simulink library "Geartrain_Lib"  (R2025a)
settings: Solver=ode45  StartTime=0.0  StopTime=10.0  RelTol=1e-3  EnableMultiTasking=on
undefined symbols (not defined in the file): WT_Params
libraries: fl_lib x8, sdl_lib x3, nesl_utility x2, Brakes_Lib x1
Description:
  | Copyright 2009-2025 The MathWorks, Inc. MathWorks, Inc.
settings Model: Creator=smiller  LastModifiedBy=smiller
settings SolverCC: AlgebraicLoopSolver=TrustRegion
settings DataIOCC: LimitDataPoints=on  SaveFormat=Array  SignalLoggingSaveFormat=ModelDataLogs  ReturnWorkspaceOutputs=off
settings OptimizationCC: ReuseModelBlockBuffer=off  ExpressionDepthLimit=2147483647.0  LifeSpan=inf
settings DebuggingCC: UnderspecifiedInitializationDetection=Classic  MergeDetectMultiDrivingBlocksExec=none  SolverPrmCheckMsg=warning  FcnCallInpInsideContextMsg=warning  UnconnectedInputMsg=warning  UnconnectedOutputMsg=warning  UnconnectedLineMsg=warning  AllowSymbolicDim=off  StateNameClashWarn=warning  PregeneratedLibrarySubsystemCodeDiagnostic=none  SFUnexpectedBacktrackingDiag=warning  SFNoUnconditionalDefaultTransitionDiag=warning  SFExecutionAtInitializationDiag=none  ArithmeticOperatorsInVariantConditions=warning
settings HardwareCC: ProdBitPerPointer=32.0  ProdBitPerSizeT=32.0  ProdBitPerPtrDiffT=32.0  ProdLargestAtomicFloat=None  ProdIntDivRoundTo=Undefined  ProdEndianess=Unspecified  ProdWordSize=32.0  ProdHWDeviceType=32-bit Generic
settings ModelReferenceCC: EnableRefExpFcnMdlSchedulingChecks=on  PropagateSignalLabelsOutOfModel=off
settings SFSimCC: SimUseLocalCustomCode=off  CustomCodeUndefinedFunction=UseInterfaceOnly
settings RTWCC: RTWUseLocalCustomCode=off  GPUComputeCapability=3.5  DLArmComputeVersion=19.05
settings CodeAppCC: StateflowObjectComments=on
settings GRTTargetCC: TargetLangStandard=C89/C90 (ANSI)  CombineOutputUpdateFcns=off  GRTInterface=on
settings ConfigComp: CovMetricSettings=dw  CovSaveCumulativeToWorkspaceVar=on  CovSaveSingleToWorkspaceVar=on  CovExternalEMLEnable=off  CovSFcnEnable=off

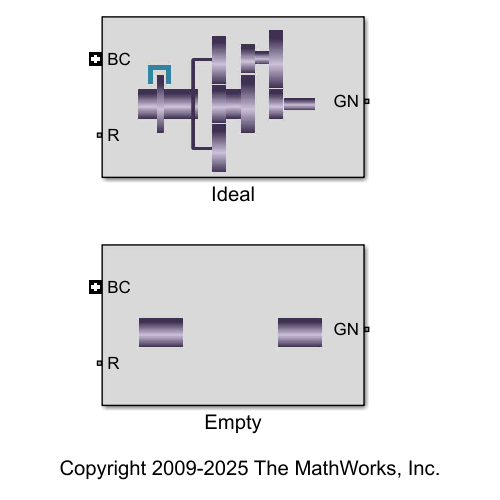
[thumbnail: Simulink's stored preview of the top-level diagram]
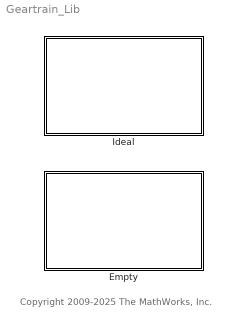
== system Geartrain_Lib ==
  note: Copyright 2009-2025 The MathWorks, Inc.
  Empty : Subsystem
      mask Display: image('Geartrain_Empty_IMAGE.jpg');
  Ideal : Subsystem
      mask Display: image('Geartrain_Ideal_IMAGE.jpg');

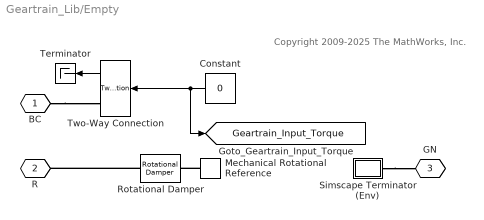
== system Geartrain_Lib/Empty ==
  note: Copyright 2009-2025 The MathWorks, Inc.
  Constant : Constant  Value=0
  Mechanical Rotational Reference : fl_lib/Mechanical/Rotational Elements/Mechanical Rotational Reference
  Rotational Damper : fl_lib/Mechanical/Rotational Elements/Rotational Damper  D=WT_Params.Empty_Geartrain.damping N*m/(rad/s)  w_specify=off  w_priority=High  w=0 rad/s  w_nominal_specify=off  w_nominal_value=1  w_nominal_unit=rad/s  t_specify=off  t_priority=High  t=0 N*m  t_nominal_specify=off  t_nominal_value=1  t_nominal_unit=N*m
  Simscape Terminator (Env) : Subsystem
      mask Display:
      | plot([0 0.9],[0.5 0.5]);
      | plot([0.5 0.9],[0.3 0.3]);
      | plot([0.5 0.9],[0.7 0.7]);
      | plot([0.9 0.9],[0.7 0.3]);
  Terminator : Terminator
  Two-Way Connection : TwoWayConnection
  BC : PMIOPort  Tag=PMCPort  Side=Left
  R : PMIOPort  Tag=PMCPort  Port=2  Side=Left
  GN : PMIOPort  Tag=PMCPort  Port=3  Side=Right
  tag scope: Geartrain_Input_Torque=global
  wires:
  Two-Way Connection/1 -> Terminator/1
  Constant/1 -> Two-Way Connection/1, [Geartrain_Input_Torque]
  connections:
  BC/RConn1 -- Two-Way Connection/RConn1
  Simscape Terminator (Env)/LConn1 -- GN/RConn1
  Rotational Damper/LConn1 -- R/RConn1
  Mechanical Rotational Reference/LConn1 -- Rotational Damper/RConn1

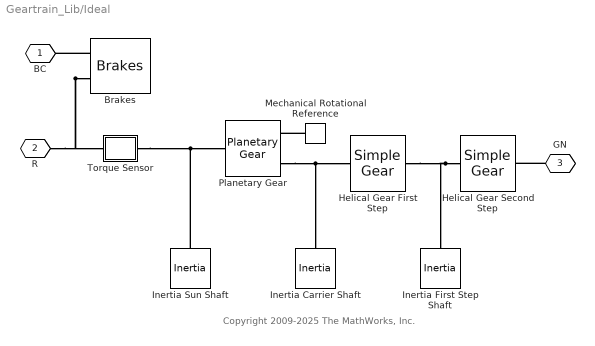
== system Geartrain_Lib/Ideal ==
  note: Copyright 2009-2025 The MathWorks, Inc.
  Brakes : Brakes_Lib/Brakes  SystemSampleTime=-1  VariantActivationTime=update diagram  EmptyChoice=off  PassThrough=off  PassThroughVariantControl=(default)  EmptyChoiceVariantControl=(default)  AllowFlexibleInterface=on  Latency=0  AutoFrameSizeCalculation=off
  Helical Gear First Step : sdl_lib/Gears/Simple Gear  ratio=WT_Params.Geartrain.Gear_Ratio.first_step  rotation_direction=3-2*(2)  friction_model=1  T_noload=0.1 N*m  T_nom=5 N*m  efficiency_nom=0.8  efficiency=0.8  temperature_TLU=[ 280 300 320 ] K  load_TLU=[ 1 5 10 ] N*m  efficiency_TLU=[ 0.95 0.9 0.85 ]  efficiency_TLU2=[ 0.85 0.8 0.75; 0.95 0.9 0.85; 0.85 0.8 0.7 ]  w_thr=0.01 rad/s  pwr_thr=0.001 W  enable_backlash=false  hardstop_model=simscape.enum.hardstop.smooth  backlash_distance=1e-3 mm  r_base=0.1 m  transition=1e-4 mm  backlash_stiffness=1e7 N/m  backlash_damping=1e6 N*s/m  coeff_rest=0  v_tol=0.001 m/s  f_tol=0 N  mu_visc=[ 0 0 ] N*m/(rad/s)  thermal_mass=50 J/K  temperature_specify=off  temperature_priority=High  temperature=300 K  temperature_nominal_specify=off  temperature_nominal_value=1  temperature_nominal_unit=K  x_backlash_specify=off  x_backlash_priority=None  x_backlash=0 mm  x_backlash_nominal_specify=off  x_backlash_nominal_value=1  x_backlash_nominal_unit=mm  f_hardstop_specify=off  f_hardstop_priority=None  f_hardstop=0 N  f_hardstop_nominal_specify=off  f_hardstop_nominal_value=1  f_hardstop_nominal_unit=N  v_backlash_specify=off  v_backlash_priority=None  v_backlash=0 m/s  v_backlash_nominal_specify=off  v_backlash_nominal_value=1  v_backlash_nominal_unit=m/s
  Helical Gear Second Step : sdl_lib/Gears/Simple Gear  ratio=WT_Params.Geartrain.Gear_Ratio.second_step_primary_generator  rotation_direction=3-2*(2)  friction_model=1  T_noload=0.1 N*m  T_nom=5 N*m  efficiency_nom=0.8  efficiency=0.8  temperature_TLU=[ 280 300 320 ] K  load_TLU=[ 1 5 10 ] N*m  efficiency_TLU=[ 0.95 0.9 0.85 ]  efficiency_TLU2=[ 0.85 0.8 0.75; 0.95 0.9 0.85; 0.85 0.8 0.7 ]  w_thr=0.01 rad/s  pwr_thr=0.001 W  enable_backlash=false  hardstop_model=simscape.enum.hardstop.smooth  backlash_distance=1e-3 mm  r_base=0.1 m  transition=1e-4 mm  backlash_stiffness=1e7 N/m  backlash_damping=1e6 N*s/m  coeff_rest=0  v_tol=0.001 m/s  f_tol=0 N  mu_visc=[ 0 0 ] N*m/(rad/s)  thermal_mass=50 J/K  temperature_specify=off  temperature_priority=High  temperature=300 K  temperature_nominal_specify=off  temperature_nominal_value=1  temperature_nominal_unit=K  x_backlash_specify=off  x_backlash_priority=None  x_backlash=0 mm  x_backlash_nominal_specify=off  x_backlash_nominal_value=1  x_backlash_nominal_unit=mm  f_hardstop_specify=off  f_hardstop_priority=None  f_hardstop=0 N  f_hardstop_nominal_specify=off  f_hardstop_nominal_value=1  f_hardstop_nominal_unit=N  v_backlash_specify=off  v_backlash_priority=None  v_backlash=0 m/s  v_backlash_nominal_specify=off  v_backlash_nominal_value=1  v_backlash_nominal_unit=m/s
  Inertia Carrier Shaft : fl_lib/Mechanical/Rotational Elements/Inertia  inertia=WT_Params.Geartrain.inertia_sun_shaft kg*m^2  num_ports=foundation.enum.numPorts2.one  w_specify=on  w_priority=High  w=0 rad/s  w_nominal_specify=off  w_nominal_value=1  w_nominal_unit=rad/s  t_specify=off  t_priority=High  t=0 N*m  t_nominal_specify=off  t_nominal_value=1  t_nominal_unit=N*m
  Inertia First Step Shaft : fl_lib/Mechanical/Rotational Elements/Inertia  inertia=WT_Params.Geartrain.inertia_first_step_shaft kg*m^2  num_ports=foundation.enum.numPorts2.one  w_specify=on  w_priority=High  w=0 rad/s  w_nominal_specify=off  w_nominal_value=1  w_nominal_unit=rad/s  t_specify=off  t_priority=High  t=0 N*m  t_nominal_specify=off  t_nominal_value=1  t_nominal_unit=N*m
  Inertia Sun Shaft : fl_lib/Mechanical/Rotational Elements/Inertia  inertia=WT_Params.Geartrain.inertia_sun_shaft kg*m^2  num_ports=foundation.enum.numPorts2.one  w_specify=on  w_priority=High  w=0 rad/s  w_nominal_specify=off  w_nominal_value=1  w_nominal_unit=rad/s  t_specify=off  t_priority=High  t=0 N*m  t_nominal_specify=off  t_nominal_value=1  t_nominal_unit=N*m
  Mechanical Rotational Reference : fl_lib/Mechanical/Rotational Elements/Mechanical Rotational Reference
  Planetary Gear : sdl_lib/Gears/Planetary Gear  rs_ratio=WT_Params.Geartrain.Gear_Ratio.planetary  friction_model=1  efficiency=[ 0.96 0.98 ]  temperature_TLU=[ 280 300 320 ] K  efficiency_sp_TLU=[ 0.95 0.9 0.85 ]  efficiency_rp_TLU=[ 0.95 0.9 0.85 ]  pwr_thr=[ 0.001 0.001 ] W  mu_visc=WT_Params.Geartrain.Planetary.viscous_losses N*m/(rad/s)  model_inertia=0  sun_inertia=1e-10 kg*m^2  ring_inertia=1e-10 kg*m^2  carrier_inertia=1e-10 kg*m^2  carrier_radius=0.01 m  planet_inertia=0.001 kg*m^2  planet_mass=1e-10 kg  thermal_mass=50 J/K  T_init=300 K
  Torque Sensor : Subsystem
      mask Display: disp('S');
  BC : PMIOPort  Tag=PMCPort  Side=Left
  R : PMIOPort  Tag=PMCPort  Port=2  Side=Left
  GN : PMIOPort  Tag=PMCPort  Port=3  Side=Right
  connections:
  Planetary Gear/RConn2 -- Helical Gear First Step/RConn1 -- Inertia Carrier Shaft/LConn1
  Helical Gear Second Step/RConn1 -- Helical Gear First Step/LConn1 -- Inertia First Step Shaft/LConn1
  Inertia Sun Shaft/LConn1 -- Planetary Gear/LConn1 -- Torque Sensor/RConn1
  Mechanical Rotational Reference/LConn1 -- Planetary Gear/RConn1
  Brakes/LConn2 -- R/RConn1 -- Torque Sensor/LConn1
  Brakes/LConn1 -- BC/RConn1
  GN/RConn1 -- Helical Gear Second Step/LConn1

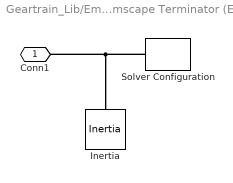
== system Geartrain_Lib/Empty/Simscape Terminator (Env) ==
  Inertia : fl_lib/Mechanical/Rotational Elements/Inertia  inertia=1.5e-3 kg*m^2  num_ports=foundation.enum.numPorts2.one  w_specify=on  w_priority=High  w=0 rad/s  w_nominal_specify=off  w_nominal_value=1  w_nominal_unit=rad/s  t_specify=off  t_priority=High  t=0 N*m  t_nominal_specify=off  t_nominal_value=1  t_nominal_unit=N*m
  Solver Configuration : nesl_utility/Solver Configuration  PhysicalDomain=network_engine_domain  SubClassName=solver  LeftPortType=input  RightPortType=generic  Tones=[]  Harmonics=[]  SimulateNoise=off  Profile=off  UseLocalSampling=off  EnableSwitchedLinearOptims=on  FrequencyDomain=off  UseCCode=off  RelTol=0.001  AbsTol=1e-06  MinStep=1e-09  ToWorkspace=off  RevertToSquareIcSolve=off  NumHomotopyIterations=100  PhasorMode=off  PhasorModeNumHarmonics=1  ConsistencySolver=NEWTON_FTOL  IndexReductionMethod=DerivativeReplacement  DoDC=off  ResidualTolerance=1e-9  ConsistencyTolSource=GLOBAL  ConsistencyAbsTol=0.001  ConsistencyRelTol=0.001  ConsistencyTolFactor=0.001  UseLocalSolver=off  LocalSolverChoice=NE_BACKWARD_EULER_ADVANCER  ResolveIndetEquations=on  FunctionEvalNumThread=1  LocalSolverSampleTime=.001  DoFixedCost=off  MaxNonlinIter=3  MaxModeIter=2  ComputeImpulses=off  ImpulseIterations=2  LinearAlgebra=Sparse  LinearAlgebraNumThread=0  EquationFormulation=NE_TIME_EF  DelaysMemoryBudget=1024  AutomaticFiltering=on  FilteringTimeConstant=0.001  PartitionStorageMethod=AS_NEEDED  PartitionMemoryBudget=1024  PartitionMethod=FAST  MultibodyUseLocalSolver=off  MultibodyLocalSolverChoice=ODE1  MultibodyLocalSolverSampleTime=0.001
  Conn1 : PMIOPort  Side=Left
  connections:
  Solver Configuration/RConn1 -- Conn1/RConn1 -- Inertia/LConn1

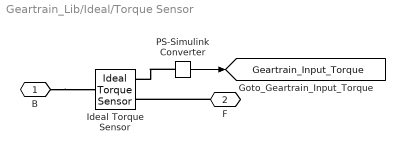
== system Geartrain_Lib/Ideal/Torque Sensor ==
  Ideal Torque Sensor : fl_lib/Mechanical/Mechanical Sensors/Ideal Torque Sensor
  PS-Simulink Converter : nesl_utility/PS-Simulink Converter  PhysicalDomain=network_engine_domain  SubClassName=ps_output  LeftPortType=input  RightPortType=output  PseudoPeriodic=off  Frequencies=[]  VectorFormat=1-D array  Unit=1  AffineConversion=off
  B : PMIOPort  Side=Left
  F : PMIOPort  Port=2  Side=Right
  tag scope: Geartrain_Input_Torque=global
  wires:
  PS-Simulink Converter/1 -> [Geartrain_Input_Torque]
  connections:
  B/RConn1 -- Ideal Torque Sensor/LConn1
  F/RConn1 -- Ideal Torque Sensor/RConn1
  PS-Simulink Converter/LConn1 -- Ideal Torque Sensor/RConn2
